simulink model "sschdlexThreePhaseConverterWithGridModel"  (R2026a)
settings: Solver=FixedStepDiscrete  StartTime=0  StopTime=0.09
InitFcn:
  | % LC filter parameters
  | 
  | Lf = 2e-3;
  | Rf = 20e-3;
  | Cf = 1e-6;
  | 
  | % Sample step size
  | 
  | % if ~exist('Tbase')
  |     Tbase = 5e-9;
  | % end
  | 
  | Ts = 1e-6;
  | Tsc=5e-5;
  | fsw = 10e3;
  | 
  | % PWM oversampling
  | oversampling = Ts/Tbase;
  | 
  | % Frame size for data transfer to CPU
  | frame_size = round(Tsc/Ts);
  | 
  | % Control constants
  | 
  | Kp_id = 1.5;
  | Ki_id = 400;
  | Kp_iq = 1.5;
  | Ki_iq = 400;
libraries: simulink x51, hdlsllib x23, fl_lib x15, nesl_utility x15, slrealtimeloglib x12, ee_lib x11, eeTransforms x3, slpidlib x2, eeSinusoidalMeasurement x1
(part 2 of 2)

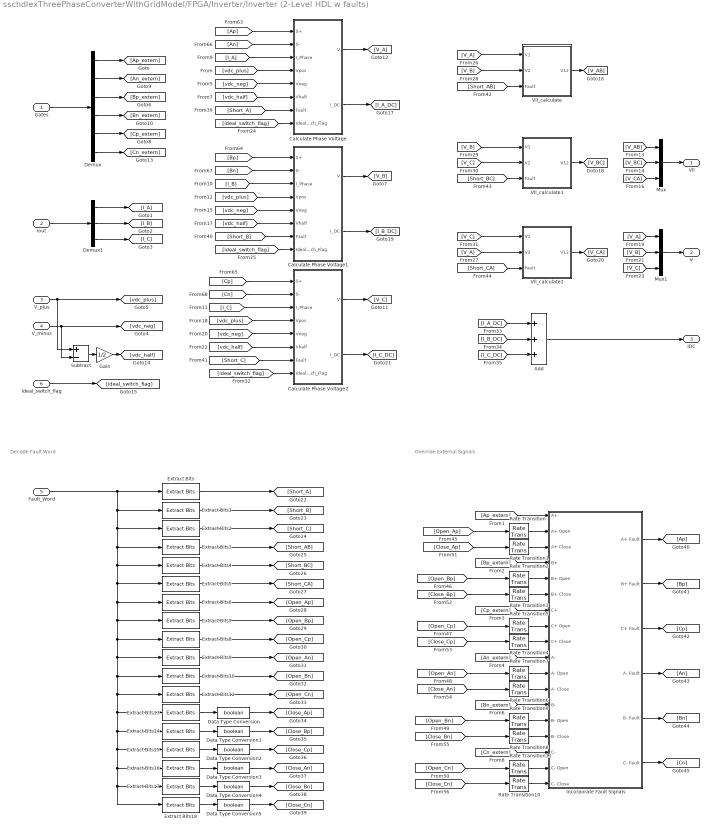
== system sschdlexThreePhaseConverterWithGridModel/FPGA/Inverter/Inverter (2-Level HDL w faults) ==
  note: Override External Signals
  note: Decode Fault Word
  Gates : Inport
  Iout : Inport  Port=2
  V_plus : Inport  Port=3
  V_minus : Inport  Port=4
  Fault_Word : Inport  Port=5
  ideal_switch_flag : Inport  Port=6
  Add : Sum  Inputs=+++
  Calculate Phase Voltage : Subsystem
  Calculate Phase Voltage1 : Subsystem
  Calculate Phase Voltage2 : Subsystem
  Data Type Conversion{,1..5} (6 alike) : DataTypeConversion  OutDataTypeStr=boolean  SaturateOnIntegerOverflow=off  RndMeth=Floor
  Demux : Demux  Outputs=6
  Demux1 : Demux  Outputs=3
  Extract Bits : simulink/Logic and Bit Operations/Extract Bits  bitsToExtract=Range of bits  numBits=8  bitIdxRange=[0]  outScalingMode=Treat bit field as an integer
  Extract Bits1 : simulink/Logic and Bit Operations/Extract Bits  bitsToExtract=Range of bits  numBits=8  bitIdxRange=1  outScalingMode=Treat bit field as an integer
  Extract Bits10 : simulink/Logic and Bit Operations/Extract Bits  bitsToExtract=Range of bits  numBits=8  bitIdxRange=10  outScalingMode=Treat bit field as an integer
  Extract Bits12 : simulink/Logic and Bit Operations/Extract Bits  bitsToExtract=Range of bits  numBits=8  bitIdxRange=11  outScalingMode=Treat bit field as an integer
  Extract Bits13 : simulink/Logic and Bit Operations/Extract Bits  bitsToExtract=Range of bits  numBits=8  bitIdxRange=12  outScalingMode=Treat bit field as an integer
  Extract Bits14 : simulink/Logic and Bit Operations/Extract Bits  bitsToExtract=Range of bits  numBits=8  bitIdxRange=13  outScalingMode=Treat bit field as an integer
  Extract Bits15 : simulink/Logic and Bit Operations/Extract Bits  bitsToExtract=Range of bits  numBits=8  bitIdxRange=14  outScalingMode=Treat bit field as an integer
  Extract Bits16 : simulink/Logic and Bit Operations/Extract Bits  bitsToExtract=Range of bits  numBits=8  bitIdxRange=15  outScalingMode=Treat bit field as an integer
  Extract Bits17 : simulink/Logic and Bit Operations/Extract Bits  bitsToExtract=Range of bits  numBits=8  bitIdxRange=16  outScalingMode=Treat bit field as an integer
  Extract Bits18 : simulink/Logic and Bit Operations/Extract Bits  bitsToExtract=Range of bits  numBits=8  bitIdxRange=17  outScalingMode=Treat bit field as an integer
  Extract Bits2 : simulink/Logic and Bit Operations/Extract Bits  bitsToExtract=Range of bits  numBits=8  bitIdxRange=2  outScalingMode=Treat bit field as an integer
  Extract Bits3 : simulink/Logic and Bit Operations/Extract Bits  bitsToExtract=Range of bits  numBits=8  bitIdxRange=3  outScalingMode=Treat bit field as an integer
  Extract Bits4 : simulink/Logic and Bit Operations/Extract Bits  bitsToExtract=Range of bits  numBits=8  bitIdxRange=4  outScalingMode=Treat bit field as an integer
  Extract Bits5 : simulink/Logic and Bit Operations/Extract Bits  bitsToExtract=Range of bits  numBits=8  bitIdxRange=5  outScalingMode=Treat bit field as an integer
  Extract Bits6 : simulink/Logic and Bit Operations/Extract Bits  bitsToExtract=Range of bits  numBits=8  bitIdxRange=6  outScalingMode=Treat bit field as an integer
  Extract Bits7 : simulink/Logic and Bit Operations/Extract Bits  bitsToExtract=Range of bits  numBits=8  bitIdxRange=7  outScalingMode=Treat bit field as an integer
  Extract Bits8 : simulink/Logic and Bit Operations/Extract Bits  bitsToExtract=Range of bits  numBits=8  bitIdxRange=8  outScalingMode=Treat bit field as an integer
  Extract Bits9 : simulink/Logic and Bit Operations/Extract Bits  bitsToExtract=Range of bits  numBits=8  bitIdxRange=9  outScalingMode=Treat bit field as an integer
  Gain : Gain  Gain=1/2
  Incorporate Fault Signals : Subsystem
  Mux : Mux  Inputs=3
  Mux1 : Mux  Inputs=3
  Rate Transition{,1..11} (12 alike) : RateTransition  OutPortSampleTime=ts_FPGA_clk
  Subtract : Sum  Inputs=+-
  Vll_calculate : Subsystem
  Vll_calculate1 : Subsystem
  Vll_calculate2 : Subsystem
  Vll : Outport  OutDataTypeStr=single  VectorParamsAs1DForOutWhenUnconnected=off
  V : Outport  Port=2  OutDataTypeStr=single  VectorParamsAs1DForOutWhenUnconnected=off
  IDC : Outport  Port=3  OutDataTypeStr=single  VectorParamsAs1DForOutWhenUnconnected=off
  wires:
  Gates/1 -> Demux/1
  Demux/1 -> [Ap_extern]
  Demux/3 -> [Bp_extern]
  Demux/5 -> [Cp_extern]
  Calculate Phase Voltage/1(V) -> [V_A]
  [V_B] -> Vll_calculate/2(V2)
  [V_A] -> Vll_calculate/1(V1)
  Vll_calculate/1(V12) -> [V_AB]
  Vll_calculate2/1(V12) -> [V_CA]
  Vll_calculate1/1(V12) -> [V_BC]
  Extract Bits9/1 -> [Open_An]
  Extract Bits12/1 -> [Open_Cn]
  [Ap_extern] -> Incorporate Fault Signals/1(A+)
  Incorporate Fault Signals/6(C- Fault) -> [Cn]
  [Open_Cn] -> Rate Transition11/1
  Incorporate Fault Signals/2(B+ Fault) -> [Bp]
  [Cn_extern] -> Incorporate Fault Signals/16(C-)
  [Close_Bn] -> Rate Transition8/1
  Incorporate Fault Signals/5(B- Fault) -> [Bn]
  Extract Bits7/1 -> [Open_Bp]
  [Bp_extern] -> Incorporate Fault Signals/4(B+)
  [Close_Cn] -> Rate Transition10/1
  [Close_Bp] -> Rate Transition3/1
  [Open_Bp] -> Rate Transition2/1
  [Bn_extern] -> Incorporate Fault Signals/13(B-)
  [Close_An] -> Rate Transition6/1
  [An_extern] -> Incorporate Fault Signals/10(A-)
  Fault_Word/1 -> Extract Bits/1, Extract Bits1/1, Extract Bits2/1, Extract Bits3/1, Extract Bits4/1, Extract Bits5/1, Extract Bits6/1, Extract Bits7/1, Extract Bits8/1, Extract Bits9/1, Extract Bits10/1, Extract Bits12/1, Extract Bits13/1, Extract Bits14/1, Extract Bits15/1, Extract Bits16/1, Extract Bits18/1, Extract Bits17/1
  Extract Bits6/1 -> [Open_Ap]
  [Open_Ap] -> Rate Transition/1
  Extract Bits8/1 -> [Open_Cp]
  Extract Bits17/1 -> Data Type Conversion4/1
  [Cp_extern] -> Incorporate Fault Signals/7(C+)
  Extract Bits5/1 -> [Short_CA]
  Extract Bits14/1 -> Data Type Conversion1/1
  Extract Bits1/1 -> [Short_B]
  Extract Bits13/1 -> Data Type Conversion/1
  Extract Bits10/1 -> [Open_Bn]
  Incorporate Fault Signals/4(A- Fault) -> [An]
  [Close_Ap] -> Rate Transition1/1
  [Open_Cp] -> Rate Transition5/1
  Incorporate Fault Signals/1(A+ Fault) -> [Ap]
  Extract Bits4/1 -> [Short_BC]
  Extract Bits18/1 -> Data Type Conversion5/1
  Extract Bits3/1 -> [Short_AB]
  [Open_Bn] -> Rate Transition9/1
  Extract Bits2/1 -> [Short_C]
  [Open_An] -> Rate Transition7/1
  Extract Bits15/1 -> Data Type Conversion2/1
  Extract Bits/1 -> [Short_A]
  Incorporate Fault Signals/3(C+ Fault) -> [Cp]
  [Close_Cp] -> Rate Transition4/1
  Extract Bits16/1 -> Data Type Conversion3/1
  Iout/1 -> Demux1/1
  Demux1/1 -> [I_A]
  Demux1/2 -> [I_B]
  Demux1/3 -> [I_C]
  [Ap] -> Calculate Phase Voltage/1(S+)
  [I_A] -> Calculate Phase Voltage/3(I_Phase)
  [An] -> Calculate Phase Voltage/2(S-)
  [vdc_plus] -> Calculate Phase Voltage/4(Vpos)
  [vdc_neg] -> Calculate Phase Voltage/5(Vneg)
  [vdc_half] -> Calculate Phase Voltage/6(Vhalf)
  [Short_A] -> Calculate Phase Voltage/7(Fault)
  [Bp] -> Calculate Phase Voltage1/1(S+)
  [Bn] -> Calculate Phase Voltage1/2(S-)
  [I_B] -> Calculate Phase Voltage1/3(I_Phase)
  [vdc_plus] -> Calculate Phase Voltage1/4(Vpos)
  [vdc_neg] -> Calculate Phase Voltage1/5(Vneg)
  [vdc_half] -> Calculate Phase Voltage1/6(Vhalf)
  [Short_B] -> Calculate Phase Voltage1/7(Fault)
  [I_C] -> Calculate Phase Voltage2/3(I_Phase)
  [Cp] -> Calculate Phase Voltage2/1(S+)
  [Cn] -> Calculate Phase Voltage2/2(S-)
  [vdc_plus] -> Calculate Phase Voltage2/4(Vpos)
  [vdc_neg] -> Calculate Phase Voltage2/5(Vneg)
  [Short_C] -> Calculate Phase Voltage2/7(Fault)
  [vdc_half] -> Calculate Phase Voltage2/6(Vhalf)
  Calculate Phase Voltage1/1(V) -> [V_B]
  Calculate Phase Voltage2/1(V) -> [V_C]
  [V_C] -> Vll_calculate2/1(V1)
  [V_A] -> Vll_calculate2/2(V2)
  [V_B] -> Vll_calculate1/1(V1)
  [V_C] -> Vll_calculate1/2(V2)
  [Short_AB] -> Vll_calculate/3(Fault)
  [Short_BC] -> Vll_calculate1/3(Fault)
  [Short_CA] -> Vll_calculate2/3(Fault)
  [V_BC] -> Mux/2
  [V_CA] -> Mux/3
  [V_AB] -> Mux/1
  Mux/1 -> Vll/1
  V_plus/1 -> Subtract/1, [vdc_plus]
  V_minus/1 -> Subtract/2, [vdc_neg]
  Subtract/1 -> Gain/1
  Gain/1 -> [vdc_half]
  Data Type Conversion/1 -> [Close_Ap]
  Data Type Conversion1/1 -> [Close_Bp]
  Data Type Conversion2/1 -> [Close_Cp]
  Data Type Conversion3/1 -> [Close_An]
  Data Type Conversion4/1 -> [Close_Bn]
  Data Type Conversion5/1 -> [Close_Cn]
  Mux1/1 -> V/1
  [V_A] -> Mux1/1
  [V_C] -> Mux1/3
  [V_B] -> Mux1/2
  ideal_switch_flag/1 -> [ideal_switch_flag]
  [ideal_switch_flag] -> Calculate Phase Voltage/8(Ideal_Switch_Flag)
  [ideal_switch_flag] -> Calculate Phase Voltage1/8(Ideal_Switch_Flag)
  [ideal_switch_flag] -> Calculate Phase Voltage2/8(Ideal_Switch_Flag)
  Demux/2 -> [An_extern]
  Demux/4 -> [Bn_extern]
  Demux/6 -> [Cn_extern]
  Calculate Phase Voltage/2(I_DC) -> [I_A_DC]
  Calculate Phase Voltage1/2(I_DC) -> [I_B_DC]
  Calculate Phase Voltage2/2(I_DC) -> [I_C_DC]
  [I_A_DC] -> Add/1
  [I_B_DC] -> Add/2
  [I_C_DC] -> Add/3
  Add/1 -> IDC/1
  Rate Transition/1 -> Incorporate Fault Signals/2(A+ Open)
  Rate Transition1/1 -> Incorporate Fault Signals/3(A+ Close)
  Rate Transition2/1 -> Incorporate Fault Signals/5(B+ Open)
  Rate Transition3/1 -> Incorporate Fault Signals/6(B+ Close)
  Rate Transition4/1 -> Incorporate Fault Signals/9(C+ Close)
  Rate Transition5/1 -> Incorporate Fault Signals/8(C+ Open)
  Rate Transition7/1 -> Incorporate Fault Signals/11(A- Open)
  Rate Transition6/1 -> Incorporate Fault Signals/12(A- Close)
  Rate Transition9/1 -> Incorporate Fault Signals/14(B- Open)
  Rate Transition8/1 -> Incorporate Fault Signals/15(B- Close)
  Rate Transition10/1 -> Incorporate Fault Signals/18(C- Close)
  Rate Transition11/1 -> Incorporate Fault Signals/17(C- Open)

== system sschdlexThreePhaseConverterWithGridModel/FPGA/PWM Generator/Carrier ==
  Enable : Inport  OutDataTypeStr=boolean  PortDimensions=1
  PWM Period : Inport  Port=2  OutDataTypeStr=uint32  PortDimensions=1
  Abs : Abs  OutDataTypeStr=uint32  SaturateOnIntegerOverflow=off
  HDL Counter : hdlsllib/Sources/HDL Counter  CountType=Free running  CountInit=0  CountStep=1  CountMax=25  CountFromType=Initial value  CountFrom=0  CountResetPort=on  CountLoadPort=off  CountEnbPort=on  CountDirPort=off  CountHitOutputPort=off  CountDataType=Unsigned  CountWordLen=32  CountFracLen=0  CountSampTime=1
  Minus : Sum  Inputs=+-  OutDataTypeStr=int32
  Multiply : Gain  Gain=2  OutDataTypeStr=uint32
  NOT : Logic  Operator=NOT  AllPortsSameDT=off  OutDataTypeStr=boolean
  OR : Logic  Operator=OR  AllPortsSameDT=off  OutDataTypeStr=boolean
  Relational Operator : RelationalOperator  OutDataTypeStr=boolean  InputSameDT=off
  Counter : Outport  VectorParamsAs1DForOutWhenUnconnected=off
  wires:
  Relational Operator/1 -> OR/1
  HDL Counter/1 -> Relational Operator/1, Minus/1
  Enable/1 -> NOT/1, HDL Counter/2
  PWM Period/1 -> Multiply/1, Minus/2
  Minus/1 -> Abs/1
  Abs/1 -> Counter/1
  Multiply/1 -> Relational Operator/2
  OR/1 -> HDL Counter/1
  NOT/1 -> OR/2

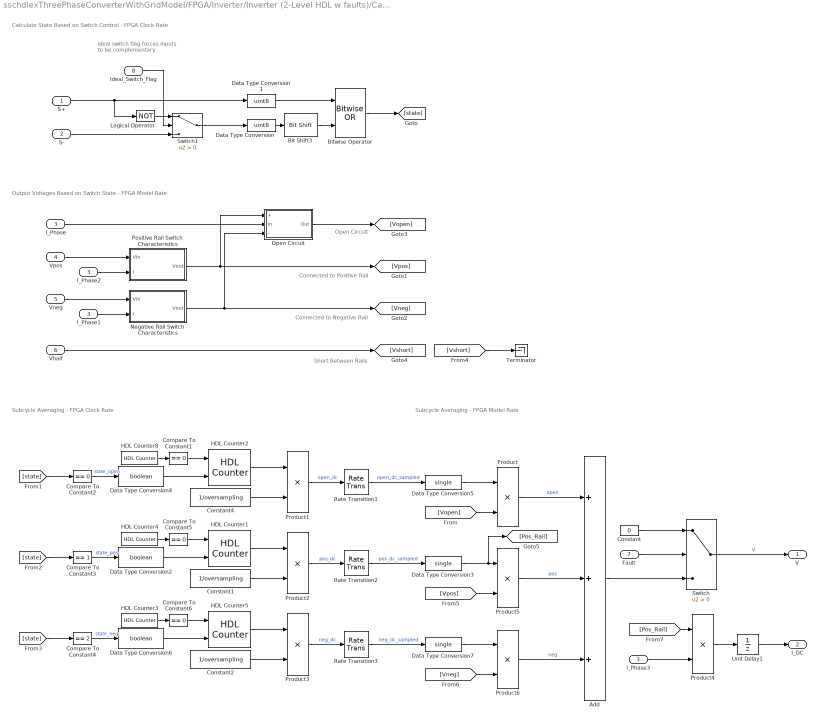
== system sschdlexThreePhaseConverterWithGridModel/FPGA/Inverter/Inverter (2-Level HDL w faults)/Calculate Phase Voltage ==
  note: Subcycle Averaging - FPGA Clock Rate
  note: ideal switch flag forces
      | inputs to be complementary
  note: Open Circuit
  note: Connected to Positive Rail
  note: Connected to Negative Rail
  note: Short Between Rails
  note: Subcycle Averaging - FPGA Model Rate
  note: Output Voltages Based on Switch State - FPGA Model Rate
  note: Calculate State Based on Switch Control - FPGA Clock Rate
  S+ : Inport
  S- : Inport  Port=2
  I_Phase : Inport  Port=3
  Vpos : Inport  Port=4
  Vneg : Inport  Port=5
  Vhalf : Inport  Port=6
  Fault : Inport  Port=7
  Ideal_Switch_Flag : Inport  Port=8
  Add : Sum  Inputs=+++
  Bit Shift3 : hdlsllib/Logic and Bit Operations/Bit Shift  mode=Shift Left Logical  N=1
  Bitwise Operator : simulink/Logic and Bit Operations/Bitwise Operator  logicop=OR  UseBitMask=off  NumInputPorts=2  BitMask=bin2dec('11011001')  BitMaskRealWorld=Stored Integer
  Compare To Constant{1..2,5..6} (4 alike) : simulink/Logic and Bit Operations/Compare To Constant  relop===  const=0  OutDataTypeStr=boolean
  Compare To Constant3 : simulink/Logic and Bit Operations/Compare To Constant  relop===  const=1  OutDataTypeStr=boolean
  Compare To Constant4 : simulink/Logic and Bit Operations/Compare To Constant  relop===  const=2  OutDataTypeStr=boolean
  Constant : Constant  Value=0  OutDataTypeStr=single  SampleTime=ts_FPGA_mdl
  Constant1 : Constant  Value=1/oversampling  OutDataTypeStr=fixdt(0,18,18)  SampleTime=ts_FPGA_clk
  Constant2 : Constant  Value=1/oversampling  OutDataTypeStr=fixdt(0,18,18)  SampleTime=ts_FPGA_clk
  Constant4 : Constant  Value=1/oversampling  OutDataTypeStr=fixdt(0,18,18)  SampleTime=ts_FPGA_clk
  Data Type Conversion : DataTypeConversion  OutDataTypeStr=uint8  SaturateOnIntegerOverflow=off  RndMeth=Floor
  Data Type Conversion1 : DataTypeConversion  OutDataTypeStr=uint8  SaturateOnIntegerOverflow=off  RndMeth=Floor
  Data Type Conversion2 : DataTypeConversion  OutDataTypeStr=boolean  SaturateOnIntegerOverflow=off  RndMeth=Floor
  Data Type Conversion3 : DataTypeConversion  OutDataTypeStr=single  SaturateOnIntegerOverflow=off  RndMeth=Floor
  Data Type Conversion4 : DataTypeConversion  OutDataTypeStr=boolean  SaturateOnIntegerOverflow=off  RndMeth=Floor
  Data Type Conversion5 : DataTypeConversion  OutDataTypeStr=single  SaturateOnIntegerOverflow=off  RndMeth=Floor
  Data Type Conversion6 : DataTypeConversion  OutDataTypeStr=boolean  SaturateOnIntegerOverflow=off  RndMeth=Floor
  Data Type Conversion7 : DataTypeConversion  OutDataTypeStr=single  SaturateOnIntegerOverflow=off  RndMeth=Floor
  HDL Counter1 : hdlsllib/Sources/HDL Counter  CountType=Count limited  CountInit=1  CountStep=1  CountMax=oversampling  CountFromType=Initial value  CountFrom=1  CountResetPort=on  CountLoadPort=off  CountEnbPort=on  CountDirPort=off  CountHitOutputPort=off  CountDataType=Unsigned  CountWordLen=8  CountFracLen=0  CountSampTime=1
  HDL Counter2 : hdlsllib/Sources/HDL Counter  CountType=Count limited  CountInit=1  CountStep=1  CountMax=oversampling  CountFromType=Initial value  CountFrom=1  CountResetPort=on  CountLoadPort=off  CountEnbPort=on  CountDirPort=off  CountHitOutputPort=off  CountDataType=Unsigned  CountWordLen=8  CountFracLen=0  CountSampTime=1
  HDL Counter3 : hdlsllib/Sources/HDL Counter  CountType=Count limited  CountInit=0  CountStep=1  CountMax=oversampling-1  CountFromType=Initial value  CountFrom=0  CountResetPort=off  CountLoadPort=off  CountEnbPort=off  CountDirPort=off  CountHitOutputPort=off  CountDataType=Unsigned  CountWordLen=8  CountFracLen=0  CountSampTime=ts_FPGA_clk
  HDL Counter4 : hdlsllib/Sources/HDL Counter  CountType=Count limited  CountInit=0  CountStep=1  CountMax=oversampling-1  CountFromType=Initial value  CountFrom=0  CountResetPort=off  CountLoadPort=off  CountEnbPort=off  CountDirPort=off  CountHitOutputPort=off  CountDataType=Unsigned  CountWordLen=8  CountFracLen=0  CountSampTime=ts_FPGA_clk
  HDL Counter5 : hdlsllib/Sources/HDL Counter  CountType=Count limited  CountInit=1  CountStep=1  CountMax=oversampling  CountFromType=Initial value  CountFrom=1  CountResetPort=on  CountLoadPort=off  CountEnbPort=on  CountDirPort=off  CountHitOutputPort=off  CountDataType=Unsigned  CountWordLen=8  CountFracLen=0  CountSampTime=1
  HDL Counter8 : hdlsllib/Sources/HDL Counter  CountType=Count limited  CountInit=0  CountStep=1  CountMax=oversampling-1  CountFromType=Initial value  CountFrom=0  CountResetPort=off  CountLoadPort=off  CountEnbPort=off  CountDirPort=off  CountHitOutputPort=off  CountDataType=Unsigned  CountWordLen=8  CountFracLen=0  CountSampTime=ts_FPGA_clk
  I_Phase1 : InportShadow  Port=3
  I_Phase2 : InportShadow  Port=3
  I_Phase3 : InportShadow  Port=3
  Logical Operator : Logic  Operator=NOT  AllPortsSameDT=off  OutDataTypeStr=boolean
  Negative Rail Switch Characteristics : Subsystem
  Open Circuit : Subsystem
  Positive Rail Switch Characteristics : Subsystem
  Product{,1..6} (7 alike) : Product
  Rate Transition1 : RateTransition  OutPortSampleTime=ts_FPGA_mdl
  Rate Transition2 : RateTransition  OutPortSampleTime=ts_FPGA_mdl
  Rate Transition3 : RateTransition  OutPortSampleTime=ts_FPGA_mdl
  Switch : Switch  Criteria=u2 > Threshold  SaturateOnIntegerOverflow=off  InputSameDT=off
  Switch1 : Switch  Criteria=u2 > Threshold  SaturateOnIntegerOverflow=off  InputSameDT=off
  Terminator : Terminator
  Unit Delay1 : UnitDelay  SampleTime=ts_FPGA_mdl
  V : Outport  VectorParamsAs1DForOutWhenUnconnected=off
  I_DC : Outport  Port=2  VectorParamsAs1DForOutWhenUnconnected=off
  wires:
  Switch/1 -> V/1  "V"
  Bit Shift3/1 -> Bitwise Operator/2
  Vpos/1 -> Positive Rail Switch Characteristics/1(Vin)
  Vhalf/1 -> [Vshort]
  Open Circuit/1(Out) -> [Vopen]
  Data Type Conversion/1 -> Bit Shift3/1
  Data Type Conversion1/1 -> Bitwise Operator/1
  Vneg/1 -> Negative Rail Switch Characteristics/1(Vin)
  S-/1 -> Switch1/3
  I_Phase/1 -> Open Circuit/2(In)
  Fault/1 -> Switch/2
  Constant/1 -> Switch/1
  Negative Rail Switch Characteristics/1(Vout) -> [Vneg], Open Circuit/3(-)
  Positive Rail Switch Characteristics/1(Vout) -> [Vpos], Open Circuit/1(+)
  I_Phase2/1 -> Positive Rail Switch Characteristics/2(I)
  I_Phase1/1 -> Negative Rail Switch Characteristics/2(I)
  Ideal_Switch_Flag/1 -> Switch1/2
  Logical Operator/1 -> Switch1/1
  Switch1/1 -> Data Type Conversion/1
  Rate Transition1/1 -> Data Type Conversion5/1  "open_dc_sampled"
  HDL Counter8/1 -> Compare To Constant1/1
  Constant4/1 -> Product1/2
  Data Type Conversion4/1 -> HDL Counter2/2
  Compare To Constant1/1 -> HDL Counter2/1
  Product1/1 -> Rate Transition1/1  "open_dc"
  HDL Counter2/1 -> Product1/1
  S+/1 -> Logical Operator/1, Data Type Conversion1/1
  Bitwise Operator/1 -> [state]
  [state] -> Compare To Constant3/1
  [state] -> Compare To Constant2/1
  [state] -> Compare To Constant4/1
  HDL Counter1/1 -> Product2/1
  Product2/1 -> Rate Transition2/1  "pos_dc"
  Compare To Constant5/1 -> HDL Counter1/1
  Data Type Conversion2/1 -> HDL Counter1/2
  Constant1/1 -> Product2/2
  HDL Counter4/1 -> Compare To Constant5/1
  Rate Transition2/1 -> Data Type Conversion3/1  "pos_dc_sampled"
  Rate Transition3/1 -> Data Type Conversion7/1  "neg_dc_sampled"
  HDL Counter3/1 -> Compare To Constant6/1
  Constant2/1 -> Product3/2
  Data Type Conversion6/1 -> HDL Counter5/2
  Compare To Constant6/1 -> HDL Counter5/1
  Product3/1 -> Rate Transition3/1  "neg_dc"
  HDL Counter5/1 -> Product3/1
  Compare To Constant4/1 -> Data Type Conversion6/1  "state_neg"
  Compare To Constant3/1 -> Data Type Conversion2/1  "state_pos"
  Compare To Constant2/1 -> Data Type Conversion4/1  "state_open"
  Add/1 -> Switch/3
  Data Type Conversion5/1 -> Product/1
  [Vopen] -> Product/2
  Data Type Conversion3/1 -> [Pos_Rail], Product5/1
  [Vpos] -> Product5/2
  Data Type Conversion7/1 -> Product6/1
  [Vneg] -> Product6/2
  Product/1 -> Add/1  "open"
  Product5/1 -> Add/2  "pos"
  Product6/1 -> Add/3  "neg"
  [Vshort] -> Terminator/1
  Product4/1 -> Unit Delay1/1
  I_Phase3/1 -> Product4/2
  [Pos_Rail] -> Product4/1
  Unit Delay1/1 -> I_DC/1

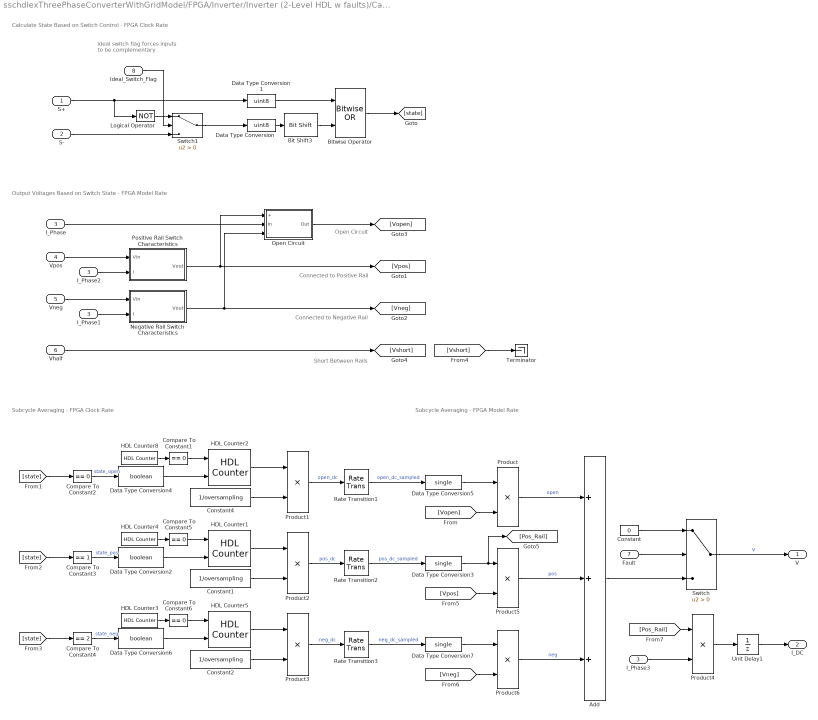
== system sschdlexThreePhaseConverterWithGridModel/FPGA/Inverter/Inverter (2-Level HDL w faults)/Calculate Phase Voltage1 ==
  note: Calculate State Based on Switch Control - FPGA Clock Rate
  note: Output Voltages Based on Switch State - FPGA Model Rate
  note: Subcycle Averaging - FPGA Model Rate
  note: Short Between Rails
  note: Connected to Negative Rail
  note: Connected to Positive Rail
  note: Open Circuit
  note: ideal switch flag forces
      | inputs to be complementary
  note: Subcycle Averaging - FPGA Clock Rate
  S+ : Inport
  S- : Inport  Port=2
  I_Phase : Inport  Port=3
  Vpos : Inport  Port=4
  Vneg : Inport  Port=5
  Vhalf : Inport  Port=6
  Fault : Inport  Port=7
  Ideal_Switch_Flag : Inport  Port=8
  Add : Sum  Inputs=+++
  Bit Shift3 : hdlsllib/Logic and Bit Operations/Bit Shift  mode=Shift Left Logical  N=1
  Bitwise Operator : simulink/Logic and Bit Operations/Bitwise Operator  logicop=OR  UseBitMask=off  NumInputPorts=2  BitMask=bin2dec('11011001')  BitMaskRealWorld=Stored Integer
  Compare To Constant{1..2,5..6} (4 alike) : simulink/Logic and Bit Operations/Compare To Constant  relop===  const=0  OutDataTypeStr=boolean
  Compare To Constant3 : simulink/Logic and Bit Operations/Compare To Constant  relop===  const=1  OutDataTypeStr=boolean
  Compare To Constant4 : simulink/Logic and Bit Operations/Compare To Constant  relop===  const=2  OutDataTypeStr=boolean
  Constant : Constant  Value=0  OutDataTypeStr=single  SampleTime=ts_FPGA_mdl
  Constant1 : Constant  Value=1/oversampling  OutDataTypeStr=fixdt(0,18,18)  SampleTime=ts_FPGA_clk
  Constant2 : Constant  Value=1/oversampling  OutDataTypeStr=fixdt(0,18,18)  SampleTime=ts_FPGA_clk
  Constant4 : Constant  Value=1/oversampling  OutDataTypeStr=fixdt(0,18,18)  SampleTime=ts_FPGA_clk
  Data Type Conversion : DataTypeConversion  OutDataTypeStr=uint8  SaturateOnIntegerOverflow=off  RndMeth=Floor
  Data Type Conversion1 : DataTypeConversion  OutDataTypeStr=uint8  SaturateOnIntegerOverflow=off  RndMeth=Floor
  Data Type Conversion2 : DataTypeConversion  OutDataTypeStr=boolean  SaturateOnIntegerOverflow=off  RndMeth=Floor
  Data Type Conversion3 : DataTypeConversion  OutDataTypeStr=single  SaturateOnIntegerOverflow=off  RndMeth=Floor
  Data Type Conversion4 : DataTypeConversion  OutDataTypeStr=boolean  SaturateOnIntegerOverflow=off  RndMeth=Floor
  Data Type Conversion5 : DataTypeConversion  OutDataTypeStr=single  SaturateOnIntegerOverflow=off  RndMeth=Floor
  Data Type Conversion6 : DataTypeConversion  OutDataTypeStr=boolean  SaturateOnIntegerOverflow=off  RndMeth=Floor
  Data Type Conversion7 : DataTypeConversion  OutDataTypeStr=single  SaturateOnIntegerOverflow=off  RndMeth=Floor
  HDL Counter1 : hdlsllib/Sources/HDL Counter  CountType=Count limited  CountInit=1  CountStep=1  CountMax=oversampling  CountFromType=Initial value  CountFrom=1  CountResetPort=on  CountLoadPort=off  CountEnbPort=on  CountDirPort=off  CountHitOutputPort=off  CountDataType=Unsigned  CountWordLen=8  CountFracLen=0  CountSampTime=1
  HDL Counter2 : hdlsllib/Sources/HDL Counter  CountType=Count limited  CountInit=1  CountStep=1  CountMax=oversampling  CountFromType=Initial value  CountFrom=1  CountResetPort=on  CountLoadPort=off  CountEnbPort=on  CountDirPort=off  CountHitOutputPort=off  CountDataType=Unsigned  CountWordLen=8  CountFracLen=0  CountSampTime=1
  HDL Counter3 : hdlsllib/Sources/HDL Counter  CountType=Count limited  CountInit=0  CountStep=1  CountMax=oversampling-1  CountFromType=Initial value  CountFrom=0  CountResetPort=off  CountLoadPort=off  CountEnbPort=off  CountDirPort=off  CountHitOutputPort=off  CountDataType=Unsigned  CountWordLen=8  CountFracLen=0  CountSampTime=ts_FPGA_clk
  HDL Counter4 : hdlsllib/Sources/HDL Counter  CountType=Count limited  CountInit=0  CountStep=1  CountMax=oversampling-1  CountFromType=Initial value  CountFrom=0  CountResetPort=off  CountLoadPort=off  CountEnbPort=off  CountDirPort=off  CountHitOutputPort=off  CountDataType=Unsigned  CountWordLen=8  CountFracLen=0  CountSampTime=ts_FPGA_clk
  HDL Counter5 : hdlsllib/Sources/HDL Counter  CountType=Count limited  CountInit=1  CountStep=1  CountMax=oversampling  CountFromType=Initial value  CountFrom=1  CountResetPort=on  CountLoadPort=off  CountEnbPort=on  CountDirPort=off  CountHitOutputPort=off  CountDataType=Unsigned  CountWordLen=8  CountFracLen=0  CountSampTime=1
  HDL Counter8 : hdlsllib/Sources/HDL Counter  CountType=Count limited  CountInit=0  CountStep=1  CountMax=oversampling-1  CountFromType=Initial value  CountFrom=0  CountResetPort=off  CountLoadPort=off  CountEnbPort=off  CountDirPort=off  CountHitOutputPort=off  CountDataType=Unsigned  CountWordLen=8  CountFracLen=0  CountSampTime=ts_FPGA_clk
  I_Phase1 : InportShadow  Port=3
  I_Phase2 : InportShadow  Port=3
  I_Phase3 : InportShadow  Port=3
  Logical Operator : Logic  Operator=NOT  AllPortsSameDT=off  OutDataTypeStr=boolean
  Negative Rail Switch Characteristics : Subsystem
  Open Circuit : Subsystem
  Positive Rail Switch Characteristics : Subsystem
  Product{,1..6} (7 alike) : Product
  Rate Transition1 : RateTransition  OutPortSampleTime=ts_FPGA_mdl
  Rate Transition2 : RateTransition  OutPortSampleTime=ts_FPGA_mdl
  Rate Transition3 : RateTransition  OutPortSampleTime=ts_FPGA_mdl
  Switch : Switch  Criteria=u2 > Threshold  SaturateOnIntegerOverflow=off  InputSameDT=off
  Switch1 : Switch  Criteria=u2 > Threshold  SaturateOnIntegerOverflow=off  InputSameDT=off
  Terminator : Terminator
  Unit Delay1 : UnitDelay  SampleTime=ts_FPGA_mdl
  V : Outport  VectorParamsAs1DForOutWhenUnconnected=off
  I_DC : Outport  Port=2  VectorParamsAs1DForOutWhenUnconnected=off
  wires:
  Unit Delay1/1 -> I_DC/1
  [Pos_Rail] -> Product4/1
  I_Phase3/1 -> Product4/2
  Product4/1 -> Unit Delay1/1
  [Vshort] -> Terminator/1
  Product6/1 -> Add/3  "neg"
  Product5/1 -> Add/2  "pos"
  Product/1 -> Add/1  "open"
  [Vneg] -> Product6/2
  Data Type Conversion7/1 -> Product6/1
  [Vpos] -> Product5/2
  Data Type Conversion3/1 -> Product5/1, [Pos_Rail]
  [Vopen] -> Product/2
  Data Type Conversion5/1 -> Product/1
  Add/1 -> Switch/3
  Compare To Constant2/1 -> Data Type Conversion4/1  "state_open"
  Compare To Constant3/1 -> Data Type Conversion2/1  "state_pos"
  Compare To Constant4/1 -> Data Type Conversion6/1  "state_neg"
  HDL Counter5/1 -> Product3/1
  Product3/1 -> Rate Transition3/1  "neg_dc"
  Compare To Constant6/1 -> HDL Counter5/1
  Data Type Conversion6/1 -> HDL Counter5/2
  Constant2/1 -> Product3/2
  HDL Counter3/1 -> Compare To Constant6/1
  Rate Transition3/1 -> Data Type Conversion7/1  "neg_dc_sampled"
  Rate Transition2/1 -> Data Type Conversion3/1  "pos_dc_sampled"
  HDL Counter4/1 -> Compare To Constant5/1
  Constant1/1 -> Product2/2
  Data Type Conversion2/1 -> HDL Counter1/2
  Compare To Constant5/1 -> HDL Counter1/1
  Product2/1 -> Rate Transition2/1  "pos_dc"
  HDL Counter1/1 -> Product2/1
  [state] -> Compare To Constant4/1
  [state] -> Compare To Constant2/1
  [state] -> Compare To Constant3/1
  Bitwise Operator/1 -> [state]
  S+/1 -> Data Type Conversion1/1, Logical Operator/1
  HDL Counter2/1 -> Product1/1
  Product1/1 -> Rate Transition1/1  "open_dc"
  Compare To Constant1/1 -> HDL Counter2/1
  Data Type Conversion4/1 -> HDL Counter2/2
  Constant4/1 -> Product1/2
  HDL Counter8/1 -> Compare To Constant1/1
  Rate Transition1/1 -> Data Type Conversion5/1  "open_dc_sampled"
  Switch1/1 -> Data Type Conversion/1
  Logical Operator/1 -> Switch1/1
  Ideal_Switch_Flag/1 -> Switch1/2
  I_Phase1/1 -> Negative Rail Switch Characteristics/2(I)
  I_Phase2/1 -> Positive Rail Switch Characteristics/2(I)
  Positive Rail Switch Characteristics/1(Vout) -> Open Circuit/1(+), [Vpos]
  Negative Rail Switch Characteristics/1(Vout) -> Open Circuit/3(-), [Vneg]
  Constant/1 -> Switch/1
  Fault/1 -> Switch/2
  I_Phase/1 -> Open Circuit/2(In)
  S-/1 -> Switch1/3
  Vneg/1 -> Negative Rail Switch Characteristics/1(Vin)
  Data Type Conversion1/1 -> Bitwise Operator/1
  Data Type Conversion/1 -> Bit Shift3/1
  Open Circuit/1(Out) -> [Vopen]
  Vhalf/1 -> [Vshort]
  Vpos/1 -> Positive Rail Switch Characteristics/1(Vin)
  Bit Shift3/1 -> Bitwise Operator/2
  Switch/1 -> V/1  "V"

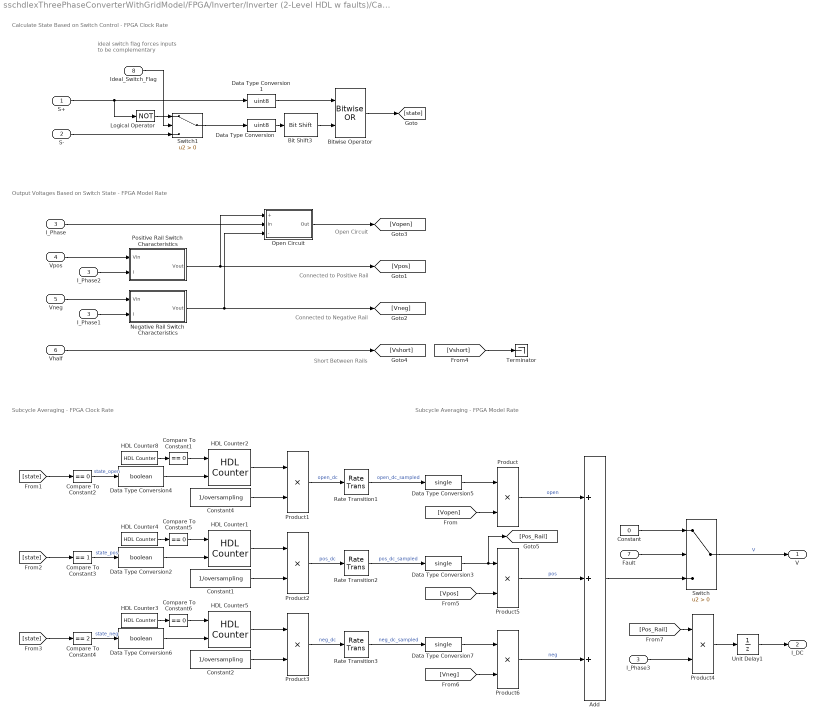
== system sschdlexThreePhaseConverterWithGridModel/FPGA/Inverter/Inverter (2-Level HDL w faults)/Calculate Phase Voltage2 ==
  note: Calculate State Based on Switch Control - FPGA Clock Rate
  note: Output Voltages Based on Switch State - FPGA Model Rate
  note: Subcycle Averaging - FPGA Model Rate
  note: Short Between Rails
  note: Connected to Negative Rail
  note: Connected to Positive Rail
  note: Open Circuit
  note: ideal switch flag forces
      | inputs to be complementary
  note: Subcycle Averaging - FPGA Clock Rate
  S+ : Inport
  S- : Inport  Port=2
  I_Phase : Inport  Port=3
  Vpos : Inport  Port=4
  Vneg : Inport  Port=5
  Vhalf : Inport  Port=6
  Fault : Inport  Port=7
  Ideal_Switch_Flag : Inport  Port=8
  Add : Sum  Inputs=+++
  Bit Shift3 : hdlsllib/Logic and Bit Operations/Bit Shift  mode=Shift Left Logical  N=1
  Bitwise Operator : simulink/Logic and Bit Operations/Bitwise Operator  logicop=OR  UseBitMask=off  NumInputPorts=2  BitMask=bin2dec('11011001')  BitMaskRealWorld=Stored Integer
  Compare To Constant{1..2,5..6} (4 alike) : simulink/Logic and Bit Operations/Compare To Constant  relop===  const=0  OutDataTypeStr=boolean
  Compare To Constant3 : simulink/Logic and Bit Operations/Compare To Constant  relop===  const=1  OutDataTypeStr=boolean
  Compare To Constant4 : simulink/Logic and Bit Operations/Compare To Constant  relop===  const=2  OutDataTypeStr=boolean
  Constant : Constant  Value=0  OutDataTypeStr=single  SampleTime=ts_FPGA_mdl
  Constant1 : Constant  Value=1/oversampling  OutDataTypeStr=fixdt(0,18,18)  SampleTime=ts_FPGA_clk
  Constant2 : Constant  Value=1/oversampling  OutDataTypeStr=fixdt(0,18,18)  SampleTime=ts_FPGA_clk
  Constant4 : Constant  Value=1/oversampling  OutDataTypeStr=fixdt(0,18,18)  SampleTime=ts_FPGA_clk
  Data Type Conversion : DataTypeConversion  OutDataTypeStr=uint8  SaturateOnIntegerOverflow=off  RndMeth=Floor
  Data Type Conversion1 : DataTypeConversion  OutDataTypeStr=uint8  SaturateOnIntegerOverflow=off  RndMeth=Floor
  Data Type Conversion2 : DataTypeConversion  OutDataTypeStr=boolean  SaturateOnIntegerOverflow=off  RndMeth=Floor
  Data Type Conversion3 : DataTypeConversion  OutDataTypeStr=single  SaturateOnIntegerOverflow=off  RndMeth=Floor
  Data Type Conversion4 : DataTypeConversion  OutDataTypeStr=boolean  SaturateOnIntegerOverflow=off  RndMeth=Floor
  Data Type Conversion5 : DataTypeConversion  OutDataTypeStr=single  SaturateOnIntegerOverflow=off  RndMeth=Floor
  Data Type Conversion6 : DataTypeConversion  OutDataTypeStr=boolean  SaturateOnIntegerOverflow=off  RndMeth=Floor
  Data Type Conversion7 : DataTypeConversion  OutDataTypeStr=single  SaturateOnIntegerOverflow=off  RndMeth=Floor
  HDL Counter1 : hdlsllib/Sources/HDL Counter  CountType=Count limited  CountInit=1  CountStep=1  CountMax=oversampling  CountFromType=Initial value  CountFrom=1  CountResetPort=on  CountLoadPort=off  CountEnbPort=on  CountDirPort=off  CountHitOutputPort=off  CountDataType=Unsigned  CountWordLen=8  CountFracLen=0  CountSampTime=1
  HDL Counter2 : hdlsllib/Sources/HDL Counter  CountType=Count limited  CountInit=1  CountStep=1  CountMax=oversampling  CountFromType=Initial value  CountFrom=1  CountResetPort=on  CountLoadPort=off  CountEnbPort=on  CountDirPort=off  CountHitOutputPort=off  CountDataType=Unsigned  CountWordLen=8  CountFracLen=0  CountSampTime=1
  HDL Counter3 : hdlsllib/Sources/HDL Counter  CountType=Count limited  CountInit=0  CountStep=1  CountMax=oversampling-1  CountFromType=Initial value  CountFrom=0  CountResetPort=off  CountLoadPort=off  CountEnbPort=off  CountDirPort=off  CountHitOutputPort=off  CountDataType=Unsigned  CountWordLen=8  CountFracLen=0  CountSampTime=ts_FPGA_clk
  HDL Counter4 : hdlsllib/Sources/HDL Counter  CountType=Count limited  CountInit=0  CountStep=1  CountMax=oversampling-1  CountFromType=Initial value  CountFrom=0  CountResetPort=off  CountLoadPort=off  CountEnbPort=off  CountDirPort=off  CountHitOutputPort=off  CountDataType=Unsigned  CountWordLen=8  CountFracLen=0  CountSampTime=ts_FPGA_clk
  HDL Counter5 : hdlsllib/Sources/HDL Counter  CountType=Count limited  CountInit=1  CountStep=1  CountMax=oversampling  CountFromType=Initial value  CountFrom=1  CountResetPort=on  CountLoadPort=off  CountEnbPort=on  CountDirPort=off  CountHitOutputPort=off  CountDataType=Unsigned  CountWordLen=8  CountFracLen=0  CountSampTime=1
  HDL Counter8 : hdlsllib/Sources/HDL Counter  CountType=Count limited  CountInit=0  CountStep=1  CountMax=oversampling-1  CountFromType=Initial value  CountFrom=0  CountResetPort=off  CountLoadPort=off  CountEnbPort=off  CountDirPort=off  CountHitOutputPort=off  CountDataType=Unsigned  CountWordLen=8  CountFracLen=0  CountSampTime=ts_FPGA_clk
  I_Phase1 : InportShadow  Port=3
  I_Phase2 : InportShadow  Port=3
  I_Phase3 : InportShadow  Port=3
  Logical Operator : Logic  Operator=NOT  AllPortsSameDT=off  OutDataTypeStr=boolean
  Negative Rail Switch Characteristics : Subsystem
  Open Circuit : Subsystem
  Positive Rail Switch Characteristics : Subsystem
  Product{,1..6} (7 alike) : Product
  Rate Transition1 : RateTransition  OutPortSampleTime=ts_FPGA_mdl
  Rate Transition2 : RateTransition  OutPortSampleTime=ts_FPGA_mdl
  Rate Transition3 : RateTransition  OutPortSampleTime=ts_FPGA_mdl
  Switch : Switch  Criteria=u2 > Threshold  SaturateOnIntegerOverflow=off  InputSameDT=off
  Switch1 : Switch  Criteria=u2 > Threshold  SaturateOnIntegerOverflow=off  InputSameDT=off
  Terminator : Terminator
  Unit Delay1 : UnitDelay  SampleTime=ts_FPGA_mdl
  V : Outport  VectorParamsAs1DForOutWhenUnconnected=off
  I_DC : Outport  Port=2  VectorParamsAs1DForOutWhenUnconnected=off
  wires:
  Unit Delay1/1 -> I_DC/1
  [Pos_Rail] -> Product4/1
  I_Phase3/1 -> Product4/2
  Product4/1 -> Unit Delay1/1
  [Vshort] -> Terminator/1
  Product6/1 -> Add/3  "neg"
  Product5/1 -> Add/2  "pos"
  Product/1 -> Add/1  "open"
  [Vneg] -> Product6/2
  Data Type Conversion7/1 -> Product6/1
  [Vpos] -> Product5/2
  Data Type Conversion3/1 -> Product5/1, [Pos_Rail]
  [Vopen] -> Product/2
  Data Type Conversion5/1 -> Product/1
  Add/1 -> Switch/3
  Compare To Constant2/1 -> Data Type Conversion4/1  "state_open"
  Compare To Constant3/1 -> Data Type Conversion2/1  "state_pos"
  Compare To Constant4/1 -> Data Type Conversion6/1  "state_neg"
  HDL Counter5/1 -> Product3/1
  Product3/1 -> Rate Transition3/1  "neg_dc"
  Compare To Constant6/1 -> HDL Counter5/1
  Data Type Conversion6/1 -> HDL Counter5/2
  Constant2/1 -> Product3/2
  HDL Counter3/1 -> Compare To Constant6/1
  Rate Transition3/1 -> Data Type Conversion7/1  "neg_dc_sampled"
  Rate Transition2/1 -> Data Type Conversion3/1  "pos_dc_sampled"
  HDL Counter4/1 -> Compare To Constant5/1
  Constant1/1 -> Product2/2
  Data Type Conversion2/1 -> HDL Counter1/2
  Compare To Constant5/1 -> HDL Counter1/1
  Product2/1 -> Rate Transition2/1  "pos_dc"
  HDL Counter1/1 -> Product2/1
  [state] -> Compare To Constant4/1
  [state] -> Compare To Constant2/1
  [state] -> Compare To Constant3/1
  Bitwise Operator/1 -> [state]
  S+/1 -> Data Type Conversion1/1, Logical Operator/1
  HDL Counter2/1 -> Product1/1
  Product1/1 -> Rate Transition1/1  "open_dc"
  Compare To Constant1/1 -> HDL Counter2/1
  Data Type Conversion4/1 -> HDL Counter2/2
  Constant4/1 -> Product1/2
  HDL Counter8/1 -> Compare To Constant1/1
  Rate Transition1/1 -> Data Type Conversion5/1  "open_dc_sampled"
  Switch1/1 -> Data Type Conversion/1
  Logical Operator/1 -> Switch1/1
  Ideal_Switch_Flag/1 -> Switch1/2
  I_Phase1/1 -> Negative Rail Switch Characteristics/2(I)
  I_Phase2/1 -> Positive Rail Switch Characteristics/2(I)
  Positive Rail Switch Characteristics/1(Vout) -> Open Circuit/1(+), [Vpos]
  Negative Rail Switch Characteristics/1(Vout) -> Open Circuit/3(-), [Vneg]
  Constant/1 -> Switch/1
  Fault/1 -> Switch/2
  I_Phase/1 -> Open Circuit/2(In)
  S-/1 -> Switch1/3
  Vneg/1 -> Negative Rail Switch Characteristics/1(Vin)
  Data Type Conversion1/1 -> Bitwise Operator/1
  Data Type Conversion/1 -> Bit Shift3/1
  Open Circuit/1(Out) -> [Vopen]
  Vhalf/1 -> [Vshort]
  Vpos/1 -> Positive Rail Switch Characteristics/1(Vin)
  Bit Shift3/1 -> Bitwise Operator/2
  Switch/1 -> V/1  "V"

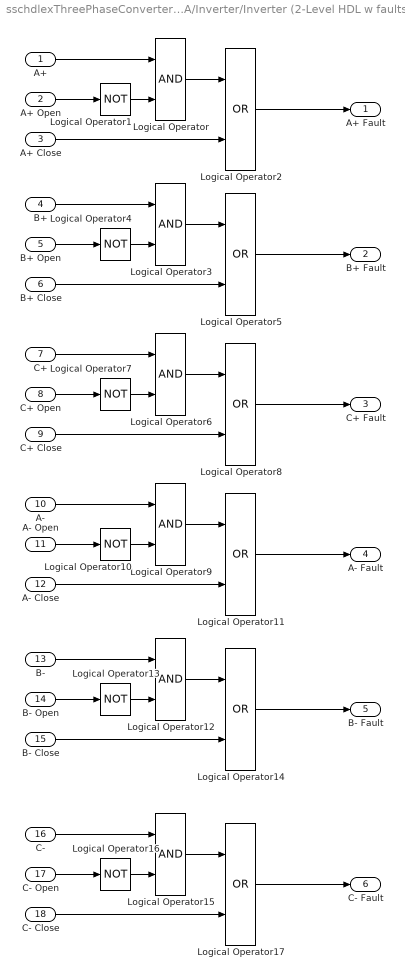
== system sschdlexThreePhaseConverterWithGridModel/FPGA/Inverter/Inverter (2-Level HDL w faults)/Incorporate Fault Signals ==
  A+ : Inport
  A+ Open : Inport  Port=2
  A+ Close : Inport  Port=3
  B+ : Inport  Port=4
  B+ Open : Inport  Port=5
  B+ Close : Inport  Port=6
  C+ : Inport  Port=7
  C+ Open : Inport  Port=8
  C+ Close : Inport  Port=9
  A- : Inport  Port=10
  A- Open : Inport  Port=11
  A- Close : Inport  Port=12
  B- : Inport  Port=13
  B- Open : Inport  Port=14
  B- Close : Inport  Port=15
  C- : Inport  Port=16
  C- Open : Inport  Port=17
  C- Close : Inport  Port=18
  Logical Operator{,3,6,9,12,15} (6 alike) : Logic  AllPortsSameDT=off  OutDataTypeStr=boolean
  Logical Operator{1,4,7,10,13,16} (6 alike) : Logic  Operator=NOT  AllPortsSameDT=off  OutDataTypeStr=boolean
  Logical Operator{2,5,8,11,14,17} (6 alike) : Logic  Operator=OR  AllPortsSameDT=off  OutDataTypeStr=boolean
  A+ Fault : Outport  VectorParamsAs1DForOutWhenUnconnected=off
  B+ Fault : Outport  Port=2  VectorParamsAs1DForOutWhenUnconnected=off
  C+ Fault : Outport  Port=3  VectorParamsAs1DForOutWhenUnconnected=off
  A- Fault : Outport  Port=4  VectorParamsAs1DForOutWhenUnconnected=off
  B- Fault : Outport  Port=5  VectorParamsAs1DForOutWhenUnconnected=off
  C- Fault : Outport  Port=6  VectorParamsAs1DForOutWhenUnconnected=off
  wires:
  Logical Operator1/1 -> Logical Operator/2
  A+ Open/1 -> Logical Operator1/1
  A+/1 -> Logical Operator/1
  A+ Close/1 -> Logical Operator2/2
  Logical Operator/1 -> Logical Operator2/1
  Logical Operator2/1 -> A+ Fault/1
  Logical Operator5/1 -> B+ Fault/1
  Logical Operator3/1 -> Logical Operator5/1
  B+ Close/1 -> Logical Operator5/2
  B+/1 -> Logical Operator3/1
  B+ Open/1 -> Logical Operator4/1
  Logical Operator4/1 -> Logical Operator3/2
  Logical Operator7/1 -> Logical Operator6/2
  C+/1 -> Logical Operator6/1
  C+ Close/1 -> Logical Operator8/2
  Logical Operator6/1 -> Logical Operator8/1
  Logical Operator8/1 -> C+ Fault/1
  Logical Operator11/1 -> A- Fault/1
  Logical Operator9/1 -> Logical Operator11/1
  A- Close/1 -> Logical Operator11/2
  A-/1 -> Logical Operator9/1
  Logical Operator10/1 -> Logical Operator9/2
  Logical Operator14/1 -> B- Fault/1
  Logical Operator12/1 -> Logical Operator14/1
  Logical Operator13/1 -> Logical Operator12/2
  B-/1 -> Logical Operator12/1
  B- Close/1 -> Logical Operator14/2
  Logical Operator17/1 -> C- Fault/1
  Logical Operator15/1 -> Logical Operator17/1
  Logical Operator16/1 -> Logical Operator15/2
  C-/1 -> Logical Operator15/1
  C- Close/1 -> Logical Operator17/2
  A- Open/1 -> Logical Operator10/1
  B- Open/1 -> Logical Operator13/1
  C- Open/1 -> Logical Operator16/1
  C+ Open/1 -> Logical Operator7/1

== system sschdlexThreePhaseConverterWithGridModel/FPGA/Inverter/Inverter (2-Level HDL w faults)/Vll_calculate ==
  V1 : Inport
  V2 : Inport  Port=2
  Fault : Inport  Port=3
  Constant : Constant  Value=0  OutDataTypeStr=single  SampleTime=-1
  Subtract2 : Sum  Inputs=+-
  Switch : Switch  Criteria=u2 > Threshold  SaturateOnIntegerOverflow=off  InputSameDT=off
  V12 : Outport  VectorParamsAs1DForOutWhenUnconnected=off
  wires:
  V2/1 -> Subtract2/2
  V1/1 -> Subtract2/1
  Subtract2/1 -> Switch/3  "V"
  Fault/1 -> Switch/2
  Switch/1 -> V12/1  "V"
  Constant/1 -> Switch/1

== system sschdlexThreePhaseConverterWithGridModel/FPGA/Inverter/Inverter (2-Level HDL w faults)/Vll_calculate1 ==
  V1 : Inport
  V2 : Inport  Port=2
  Fault : Inport  Port=3
  Constant : Constant  Value=0  OutDataTypeStr=single  SampleTime=-1
  Subtract2 : Sum  Inputs=+-
  Switch : Switch  Criteria=u2 > Threshold  SaturateOnIntegerOverflow=off  InputSameDT=off
  V12 : Outport  VectorParamsAs1DForOutWhenUnconnected=off
  wires:
  Constant/1 -> Switch/1
  Switch/1 -> V12/1  "V"
  Fault/1 -> Switch/2
  Subtract2/1 -> Switch/3  "V"
  V1/1 -> Subtract2/1
  V2/1 -> Subtract2/2

== system sschdlexThreePhaseConverterWithGridModel/FPGA/Inverter/Inverter (2-Level HDL w faults)/Vll_calculate2 ==
  V1 : Inport
  V2 : Inport  Port=2
  Fault : Inport  Port=3
  Constant : Constant  Value=0  OutDataTypeStr=single  SampleTime=-1
  Subtract2 : Sum  Inputs=+-
  Switch : Switch  Criteria=u2 > Threshold  SaturateOnIntegerOverflow=off  InputSameDT=off
  V12 : Outport  VectorParamsAs1DForOutWhenUnconnected=off
  wires:
  V2/1 -> Subtract2/2
  V1/1 -> Subtract2/1
  Subtract2/1 -> Switch/3  "V"
  Fault/1 -> Switch/2
  Switch/1 -> V12/1  "V"
  Constant/1 -> Switch/1

== system sschdlexThreePhaseConverterWithGridModel/FPGA/Inverter/Inverter (2-Level HDL w faults)/Calculate Phase Voltage/Negative Rail Switch Characteristics ==
  Vin : Inport
  I : Inport  Port=2
  Compare To Zero : simulink/Logic and Bit Operations/Compare To Zero  relop=>=  OutDataTypeStr=boolean
  Constant : Constant  Value=vfSwitch  OutDataTypeStr=single  SampleTime=ts_FPGA_mdl
  Constant1 : Constant  Value=vfDiode  OutDataTypeStr=single  SampleTime=ts_FPGA_mdl
  Gain : Gain  Gain=rSwitch
  Gain1 : Gain  Gain=rDiode
  I1 : InportShadow  Port=2
  I2 : InportShadow  Port=2
  Sum1 : Sum  Inputs=+-|
  Sum2 : Sum  Inputs=|--
  Sum3 : Sum  Inputs=++|
  Switch : Switch  Criteria=u2 > Threshold  SaturateOnIntegerOverflow=off  InputSameDT=off
  Unit Delay : UnitDelay  SampleTime=ts_FPGA_mdl
  Vout : Outport  VectorParamsAs1DForOutWhenUnconnected=off
  wires:
  I/1 -> Gain/1
  Gain1/1 -> Sum2/1
  Sum3/1 -> Unit Delay/1
  Switch/1 -> Sum3/2
  I1/1 -> Compare To Zero/1
  Vin/1 -> Sum3/1
  Unit Delay/1 -> Vout/1
  Constant/1 -> Sum1/1
  I2/1 -> Gain1/1
  Sum1/1 -> Switch/3
  Gain/1 -> Sum1/2
  Sum2/1 -> Switch/1
  Constant1/1 -> Sum2/2
  Compare To Zero/1 -> Switch/2

== system sschdlexThreePhaseConverterWithGridModel/FPGA/Inverter/Inverter (2-Level HDL w faults)/Calculate Phase Voltage/Open Circuit ==
  + : Inport
  In : Inport  Port=2
  - : Inport  Port=3
  Gain : Gain  Gain=-rSnub
  Max : MinMax  Inputs=2
  Max1 : MinMax  Function=max  Inputs=2
  Unit Delay : UnitDelay  SampleTime=ts_FPGA_mdl
  Out : Outport  VectorParamsAs1DForOutWhenUnconnected=off
  wires:
  -/1 -> Max1/2
  Max/1 -> Unit Delay/1
  +/1 -> Max/1
  Gain/1 -> Max1/1
  In/1 -> Gain/1
  Max1/1 -> Max/2
  Unit Delay/1 -> Out/1

== system sschdlexThreePhaseConverterWithGridModel/FPGA/Inverter/Inverter (2-Level HDL w faults)/Calculate Phase Voltage/Positive Rail Switch Characteristics ==
  Vin : Inport
  I : Inport  Port=2
  Compare To Zero : simulink/Logic and Bit Operations/Compare To Zero  relop=>=  OutDataTypeStr=boolean
  Constant : Constant  Value=vfSwitch  OutDataTypeStr=single  SampleTime=ts_FPGA_mdl
  Constant1 : Constant  Value=vfDiode  OutDataTypeStr=single  SampleTime=ts_FPGA_mdl
  Gain : Gain  Gain=rSwitch
  Gain1 : Gain  Gain=rDiode
  I1 : InportShadow  Port=2
  I2 : InportShadow  Port=2
  Sum1 : Sum  Inputs=-+|
  Sum2 : Sum  Inputs=|++
  Sum3 : Sum  Inputs=+-|
  Switch : Switch  Criteria=u2 > Threshold  SaturateOnIntegerOverflow=off  InputSameDT=off
  Unit Delay : UnitDelay  SampleTime=ts_FPGA_mdl
  Vout : Outport  VectorParamsAs1DForOutWhenUnconnected=off
  wires:
  I/1 -> Gain/1
  Constant/1 -> Sum2/2
  Sum2/1 -> Switch/1
  Unit Delay/1 -> Vout/1
  Gain/1 -> Sum2/1
  Vin/1 -> Sum3/1
  I1/1 -> Compare To Zero/1
  Switch/1 -> Sum3/2
  Gain1/1 -> Sum1/2
  Constant1/1 -> Sum1/1
  I2/1 -> Gain1/1
  Sum1/1 -> Switch/3
  Sum3/1 -> Unit Delay/1
  Compare To Zero/1 -> Switch/2

== system sschdlexThreePhaseConverterWithGridModel/FPGA/Inverter/Inverter (2-Level HDL w faults)/Calculate Phase Voltage1/Negative Rail Switch Characteristics ==
  Vin : Inport
  I : Inport  Port=2
  Compare To Zero : simulink/Logic and Bit Operations/Compare To Zero  relop=>=  OutDataTypeStr=boolean
  Constant : Constant  Value=vfSwitch  OutDataTypeStr=single  SampleTime=ts_FPGA_mdl
  Constant1 : Constant  Value=vfDiode  OutDataTypeStr=single  SampleTime=ts_FPGA_mdl
  Gain : Gain  Gain=rSwitch
  Gain1 : Gain  Gain=rDiode
  I1 : InportShadow  Port=2
  I2 : InportShadow  Port=2
  Sum1 : Sum  Inputs=+-|
  Sum2 : Sum  Inputs=|--
  Sum3 : Sum  Inputs=++|
  Switch : Switch  Criteria=u2 > Threshold  SaturateOnIntegerOverflow=off  InputSameDT=off
  Unit Delay : UnitDelay  SampleTime=ts_FPGA_mdl
  Vout : Outport  VectorParamsAs1DForOutWhenUnconnected=off
  wires:
  Compare To Zero/1 -> Switch/2
  Constant1/1 -> Sum2/2
  Sum2/1 -> Switch/1
  Gain/1 -> Sum1/2
  Sum1/1 -> Switch/3
  I2/1 -> Gain1/1
  Constant/1 -> Sum1/1
  Unit Delay/1 -> Vout/1
  Vin/1 -> Sum3/1
  I1/1 -> Compare To Zero/1
  Switch/1 -> Sum3/2
  Sum3/1 -> Unit Delay/1
  Gain1/1 -> Sum2/1
  I/1 -> Gain/1

== system sschdlexThreePhaseConverterWithGridModel/FPGA/Inverter/Inverter (2-Level HDL w faults)/Calculate Phase Voltage1/Open Circuit ==
  + : Inport
  In : Inport  Port=2
  - : Inport  Port=3
  Gain : Gain  Gain=-rSnub
  Max : MinMax  Inputs=2
  Max1 : MinMax  Function=max  Inputs=2
  Unit Delay : UnitDelay  SampleTime=ts_FPGA_mdl
  Out : Outport  VectorParamsAs1DForOutWhenUnconnected=off
  wires:
  Unit Delay/1 -> Out/1
  Max1/1 -> Max/2
  In/1 -> Gain/1
  Gain/1 -> Max1/1
  +/1 -> Max/1
  Max/1 -> Unit Delay/1
  -/1 -> Max1/2

== system sschdlexThreePhaseConverterWithGridModel/FPGA/Inverter/Inverter (2-Level HDL w faults)/Calculate Phase Voltage1/Positive Rail Switch Characteristics ==
  Vin : Inport
  I : Inport  Port=2
  Compare To Zero : simulink/Logic and Bit Operations/Compare To Zero  relop=>=  OutDataTypeStr=boolean
  Constant : Constant  Value=vfSwitch  OutDataTypeStr=single  SampleTime=ts_FPGA_mdl
  Constant1 : Constant  Value=vfDiode  OutDataTypeStr=single  SampleTime=ts_FPGA_mdl
  Gain : Gain  Gain=rSwitch
  Gain1 : Gain  Gain=rDiode
  I1 : InportShadow  Port=2
  I2 : InportShadow  Port=2
  Sum1 : Sum  Inputs=-+|
  Sum2 : Sum  Inputs=|++
  Sum3 : Sum  Inputs=+-|
  Switch : Switch  Criteria=u2 > Threshold  SaturateOnIntegerOverflow=off  InputSameDT=off
  Unit Delay : UnitDelay  SampleTime=ts_FPGA_mdl
  Vout : Outport  VectorParamsAs1DForOutWhenUnconnected=off
  wires:
  Compare To Zero/1 -> Switch/2
  Sum3/1 -> Unit Delay/1
  Sum1/1 -> Switch/3
  I2/1 -> Gain1/1
  Constant1/1 -> Sum1/1
  Gain1/1 -> Sum1/2
  Switch/1 -> Sum3/2
  I1/1 -> Compare To Zero/1
  Vin/1 -> Sum3/1
  Gain/1 -> Sum2/1
  Unit Delay/1 -> Vout/1
  Sum2/1 -> Switch/1
  Constant/1 -> Sum2/2
  I/1 -> Gain/1

== system sschdlexThreePhaseConverterWithGridModel/FPGA/Inverter/Inverter (2-Level HDL w faults)/Calculate Phase Voltage2/Negative Rail Switch Characteristics ==
  Vin : Inport
  I : Inport  Port=2
  Compare To Zero : simulink/Logic and Bit Operations/Compare To Zero  relop=>=  OutDataTypeStr=boolean
  Constant : Constant  Value=vfSwitch  OutDataTypeStr=single  SampleTime=ts_FPGA_mdl
  Constant1 : Constant  Value=vfDiode  OutDataTypeStr=single  SampleTime=ts_FPGA_mdl
  Gain : Gain  Gain=rSwitch
  Gain1 : Gain  Gain=rDiode
  I1 : InportShadow  Port=2
  I2 : InportShadow  Port=2
  Sum1 : Sum  Inputs=+-|
  Sum2 : Sum  Inputs=|--
  Sum3 : Sum  Inputs=++|
  Switch : Switch  Criteria=u2 > Threshold  SaturateOnIntegerOverflow=off  InputSameDT=off
  Unit Delay : UnitDelay  SampleTime=ts_FPGA_mdl
  Vout : Outport  VectorParamsAs1DForOutWhenUnconnected=off
  wires:
  Compare To Zero/1 -> Switch/2
  Constant1/1 -> Sum2/2
  Sum2/1 -> Switch/1
  Gain/1 -> Sum1/2
  Sum1/1 -> Switch/3
  I2/1 -> Gain1/1
  Constant/1 -> Sum1/1
  Unit Delay/1 -> Vout/1
  Vin/1 -> Sum3/1
  I1/1 -> Compare To Zero/1
  Switch/1 -> Sum3/2
  Sum3/1 -> Unit Delay/1
  Gain1/1 -> Sum2/1
  I/1 -> Gain/1

== system sschdlexThreePhaseConverterWithGridModel/FPGA/Inverter/Inverter (2-Level HDL w faults)/Calculate Phase Voltage2/Open Circuit ==
  + : Inport
  In : Inport  Port=2
  - : Inport  Port=3
  Gain : Gain  Gain=-rSnub
  Max : MinMax  Inputs=2
  Max1 : MinMax  Function=max  Inputs=2
  Unit Delay : UnitDelay  SampleTime=ts_FPGA_mdl
  Out : Outport  VectorParamsAs1DForOutWhenUnconnected=off
  wires:
  Unit Delay/1 -> Out/1
  Max1/1 -> Max/2
  In/1 -> Gain/1
  Gain/1 -> Max1/1
  +/1 -> Max/1
  Max/1 -> Unit Delay/1
  -/1 -> Max1/2

== system sschdlexThreePhaseConverterWithGridModel/FPGA/Inverter/Inverter (2-Level HDL w faults)/Calculate Phase Voltage2/Positive Rail Switch Characteristics ==
  Vin : Inport
  I : Inport  Port=2
  Compare To Zero : simulink/Logic and Bit Operations/Compare To Zero  relop=>=  OutDataTypeStr=boolean
  Constant : Constant  Value=vfSwitch  OutDataTypeStr=single  SampleTime=ts_FPGA_mdl
  Constant1 : Constant  Value=vfDiode  OutDataTypeStr=single  SampleTime=ts_FPGA_mdl
  Gain : Gain  Gain=rSwitch
  Gain1 : Gain  Gain=rDiode
  I1 : InportShadow  Port=2
  I2 : InportShadow  Port=2
  Sum1 : Sum  Inputs=-+|
  Sum2 : Sum  Inputs=|++
  Sum3 : Sum  Inputs=+-|
  Switch : Switch  Criteria=u2 > Threshold  SaturateOnIntegerOverflow=off  InputSameDT=off
  Unit Delay : UnitDelay  SampleTime=ts_FPGA_mdl
  Vout : Outport  VectorParamsAs1DForOutWhenUnconnected=off
  wires:
  Compare To Zero/1 -> Switch/2
  Sum3/1 -> Unit Delay/1
  Sum1/1 -> Switch/3
  I2/1 -> Gain1/1
  Constant1/1 -> Sum1/1
  Gain1/1 -> Sum1/2
  Switch/1 -> Sum3/2
  I1/1 -> Compare To Zero/1
  Vin/1 -> Sum3/1
  Gain/1 -> Sum2/1
  Unit Delay/1 -> Vout/1
  Sum2/1 -> Switch/1
  Constant/1 -> Sum2/2
  I/1 -> Gain/1
